simulink model "NearSpace_CMG_AttitudeValidation_S07_sequential"  (R2024a)
settings: Solver=ode4  StartTime=0.0  StopTime=90  FixedStep=.001  RelTol=1e-3
InitFcn:
  | init_paths;
model workspace (MAT data in the model file):
  disturbance_schedule = [0 0.2 0.4 0.6 0.8 1 1.2 1.4 1.6 1.8 2 2.2 ... (1804 elements, 451x4)]
  native_controller_template.N = 22
  native_controller_template.nx = 11
  native_controller_template.nu = 7
  native_controller_template.A = [0.0129318474981 0.00454610585776 -0.104555464036 -0.0430961443461 0 0 0 0 0 0 0 0.0045632886618 ... (2662 elements, 11x11x22)]
  native_controller_template.B = [3.81382167025e-08 8.27941674815e-06 3.61487373465e-07 -8.73828707523e-07 0.000166666673675 6.80437440218e-11 5.83929378418e-08 0 0 0 0 -1.23300542093e-07 ... (1694 elements, 11x7x22)]
  native_controller_template.Q = [2.93800357151 1.03345970786 -23.6701188526 -9.7565805888 0 0 0 0 0 0 0 1.03345970786 ... (2783 elements, 11x11x23)]
  native_controller_template.q = [-8.33060992209e-17 -3.43379209732e-17 7.86467691392e-16 -3.63722284202e-18 0 0 0 0 0 0 0 -4.73641230657e-05 ... (253 elements, 11x23)]
  native_controller_template.R = [4.31034482759e-09 0 0 0 0 0 0 0 4.31034482759e-09 0 0 0 ... (1078 elements, 7x7x22)]
  native_controller_template.r = [0  0  0  0  0  0  0  0  0  0  0  0  0  0  0  0  0  0  0  0  0  0; 0  0  0  0  0  0  0  0  0  0  0  0  0  0  0  0  0  0  0  0  0  0; 0  0  0  0  0  0  0  0  0  0  0  0  0  0  0  0  0  0  0  0  0  0; 0  0  0  0  0  0  0  0  0  0  0  0  0  0  0  0  0  0  0  0  0  0; 0  0  0  0  0  0  0  0  0  0  0  0  0  0  0  0  0  0  0  0  0  0; 0  0  0  0  0  0  0  0  0  0  0  0  0  0  0  0  0  0  0  0  0  0; 0  0  0  0  0  0  0  0  0  0  0  0  0  0  0  0  0  0  0  0  0  0]
  native_controller_template.lu = [-7.49356523213  -7.33777259666  -7.18600471837  -7.03824308743  -6.89428580738  -6.75412475019  -6.61755652855  -6.29144837489  -5.98588397606  -5.69947563015  -5.43093373011  -4.94268279296  -4.51241818721  -4.13264174567  -3.79695534964  -3.2357799895  -2.79208095619  -2.43956912968  -2.15906876065  -1.93640270229  -1.76086736642  -1.62445125088; -40.0303246112  -39.1980515883  -38.3872802015  -37.5979115099  -36.8288669329  -36.0801029921  -35.3505331481  -33.6084121671  -31.9760422139  -30.4460095447  -29.0114244992  -26.4031327314  -24.1046185829  -22.0758239062  -20.2825675451  -17.2847500763  -14.9145096796  -13.0314021867  -11.5329854696  -10.3435215557  -9.40582937798  -8.69691379499; -5.88780125381  -5.76539275452  -5.64614656443  -5.53004814012  -5.41693884866  -5.30681230372  -5.199508701  -4.94328086598  -4.70319455262  -4.47815942369  -4.26716221651  -3.88353648019  -3.54547143281  -3.24707565731  -2.98332206043  -2.54239856318  -2.19377789415  -1.91680431618  -1.69641116908  -1.52145926608  -1.38353864504  -1.27635455426; -0.6  -0.6  -0.6  -0.6  -0.6  -0.6  -1  -1  -1  -1  -1  -1  -1  -1  -1  -1  -1  -1  -1  -1  -1  -1; -0.6  -0.6  -0.6  -0.6  -0.6  -0.6  -1  -1  -1  -1  -1  -1  -1  -1  -1  -1  -1  -1  -1  -1  -1  -1; -0.6  -0.6  -0.6  -0.6  -0.6  -0.6  -1  -1  -1  -1  -1  -1  -1  -1  -1  -1  -1  -1  -1  -1  -1  -1; -0.6  -0.6  -0.6  -0.6  -0.6  -0.6  -1  -1  -1  -1  -1  -1  -1  -1  -1  -1  -1  -1  -1  -1  -1  -1]
  native_controller_template.uu = [7.49356523213  7.33777259666  7.18600471837  7.03824308743  6.89428580738  6.75412475019  6.61755652855  6.29144837489  5.98588397606  5.69947563015  5.43093373011  4.94268279296  4.51241818721  4.13264174567  3.79695534964  3.2357799895  2.79208095619  2.43956912968  2.15906876065  1.93640270229  1.76086736642  1.62445125088; 34.0818590032  33.3733257413  32.683096134  32.011086058  31.356377316  30.7189329988  30.0978281232  28.6147036285  27.2250080988  25.9224307534  24.7011068974  22.480543243  20.5236931588  18.7964570949  17.2697381107  14.7174696001  12.6994777992  11.0962045903  9.8204418335  8.80771396137  8.0093423778  7.36908758731; 5.88780125381  5.76539275452  5.64614656443  5.53004814012  5.41693884866  5.30681230372  5.199508701  4.94328086598  4.70319455262  4.47815942369  4.26716221651  3.88353648019  3.54547143281  3.24707565731  2.98332206043  2.54239856318  2.19377789415  1.91680431618  1.69641116908  1.52145926608  1.38353864504  1.27635455426; 0.6  0.6  0.6  0.6  0.6  0.6  1  1  1  1  1  1  1  1  1  1  1  1  1  1  1  1; 0.6  0.6  0.6  0.6  0.6  0.6  1  1  1  1  1  1  1  1  1  1  1  1  1  1  1  1; 0.6  0.6  0.6  0.6  0.6  0.6  1  1  1  1  1  1  1  1  1  1  1  1  1  1  1  1; 0.6  0.6  0.6  0.6  0.6  0.6  1  1  1  1  1  1  1  1  1  1  1  1  1  1  1  1]
  native_controller_template.tr_J = [0  0  0  0  0  0  0  1  0  0  0; 0  0  0  0  0  0  0  0  1  0  0; 0  0  0  0  0  0  0  0  0  1  0; 0  0  0  0  0  0  0  0  0  0  1; 0  0  0  0  1  0  0  0  0  0  0; 0  0  0  0  0  1  0  0  0  0  0; 0  0  0  0  0  0  1  0  0  0  0]
  native_controller_template.tr_bound = [0.5 0.5 0.5 0.5 1 1 1]
  native_controller_template.dX_python = [3.23606232306e-13 -5.05417641364e-12 -2.92224535378e-12 -6.74312649502e-13 3.78845337087e-12 2.01635192376e-12 2.06409029592e-13 -1.11347932545e-13 5.50085421801e-15 1.26375661699e-13 9.48095246948e-15 2.09238232721e-07 ... (253 elements, 11x23)]
  native_controller_template.dU_python = [-0.246446738654 -0.306453966669 0.13796942633 0.00603294344725 -0.0229922476874 0.00440926582071 0.0232611456455 -0.246916325329 -0.301698755455 0.137744299807 0.00603262858184 -0.0229919425529 ... (154 elements, 7x22)]
  native_controller_template.status_python = 0
  native_controller_template.objective_python = -100.014666684
  native_controller_template.residuals_python = [2.98405715596e-07 5.55111512313e-17 5.130568831e-12 1.67492029611e-07]
  native_controller_template.time_python = 0.00536040001316
  native_controller_template.b = [0  0  0  0  0  0  0  0  0  0  0  0  0  0  0  0  0  0  0  0  0  0; 0  0  0  0  0  0  0  0  0  0  0  0  0  0  0  0  0  0  0  0  0  0; 0  0  0  0  0  0  0  0  0  0  0  0  0  0  0  0  0  0  0  0  0  0; 0  0  0  0  0  0  0  0  0  0  0  0  0  0  0  0  0  0  0  0  0  0; 0  0  0  0  0  0  0  0  0  0  0  0  0  0  0  0  0  0  0  0  0  0; 0  0  0  0  0  0  0  0  0  0  0  0  0  0  0  0  0  0  0  0  0  0; 0  0  0  0  0  0  0  0  0  0  0  0  0  0  0  0  0  0  0  0  0  0; 0  0  0  0  0  0  0  0  0  0  0  0  0  0  0  0  0  0  0  0  0  0; 0  0  0  0  0  0  0  0  0  0  0  0  0  0  0  0  0  0  0  0  0  0; 0  0  0  0  0  0  0  0  0  0  0  0  0  0  0  0  0  0  0  0  0  0; 0  0  0  0  0  0  0  0  0  0  0  0  0  0  0  0  0  0  0  0  0  0]
  native_controller_template.dts = [0.2 0.2 0.2 0.2 0.2 0.2 0.5 0.5 0.5 0.5 1 1 1 1 2 2 2 2 2 2 2 2]
  native_controller_template.X_nom = [0.99349030067 -0.00459465233533 0.105234839865 0.0433767232977 0 -0.00432732065041 -6.93889390391e-15 0 0 0 0 0.993535677662 ... (253 elements, 11x23)]
  native_controller_template.U_nom = [0  0  0  0  0  0  0  0  0  0  0  0  0  0  0  0  0  0  0  0  0  0; 0  0  0  0  0  0  0  0  0  0  0  0  0  0  0  0  0  0  0  0  0  0; 0  0  0  0  0  0  0  0  0  0  0  0  0  0  0  0  0  0  0  0  0  0; 0  0  0  0  0  0  0  0  0  0  0  0  0  0  0  0  0  0  0  0  0  0; 0  0  0  0  0  0  0  0  0  0  0  0  0  0  0  0  0  0  0  0  0  0; 0  0  0  0  0  0  0  0  0  0  0  0  0  0  0  0  0  0  0  0  0  0; 0  0  0  0  0  0  0  0  0  0  0  0  0  0  0  0  0  0  0  0  0  0]
  native_controller_template.q_ref = [0.99349030067  0.99353588687  0.993581565542  0.993627332245  0.993673182524  0.993719111908  0.993765115914  0.993880422829  0.993996097282  0.994112068092  0.99422826362  0.994461040259  0.994693846693  0.994926098112  0.995157206991  0.995613643427  0.996058465484  0.996487049594  0.996894897629  0.997277696515  0.997631377894  0.997927911665  0.997867448535; -0.00459465233533  -0.00457582315754  -0.0045568768741  -0.00453781386592  -0.00451863451821  -0.00449933922046  -0.00447992836644  -0.00443089829597  -0.00438115483786  -0.00433070450158  -0.00427955396824  -0.00417517990016  -0.00406808955824  -0.00395834267937  -0.00384600183703  -0.00361380283738  -0.00337205036695  -0.00312134796667  -0.00286234432899  -0.00259573213135  -0.00232224625292  -0.0020651359066  -0.00212009923104; 0.105234839865  0.104803580791  0.104369639557  0.103933024888  0.103493745604  0.103051810628  0.102607228979  0.10148425574  0.100344943238  0.0991894405636  0.0980179007403  0.0956273415558  0.0931745694718  0.0906609526886  0.0880879243743  0.0827696929255  0.0772326510222  0.0714906220237  0.06555846343  0.059452040163  0.0531881837227  0.0472993886305  0.0485582557271; 0.0433767232977  0.0433787136342  0.0433807080081  0.0433827062255  0.0433847080919  0.0433867134121  0.0433887219904  0.043393756399  0.0433988068547  0.0434038702496  0.0434089434559  0.0434191067035  0.0434292712519  0.0434394115678  0.0434495019994  0.0434694304446  0.043488851795  0.0435075641814  0.0435253712112  0.0435420845715  0.043557526634  0.043570473578  0.0435678337008]
  native_controller_template.omega_ref = [0  -8.67361737988e-16  -8.67361737988e-16  -8.67361737988e-16  8.67361737988e-16  0  0  0  -1.73472347598e-15  -1.73472347598e-15  8.67361737988e-16  -8.67361737988e-16  -8.67361737988e-16  0  0  0  -4.33680868994e-16  4.33680868994e-16  8.67361737988e-16  0  -4.33680868994e-16  4.33680868994e-16  4.33680868994e-16; -0.00432732065041  -0.00435416179159  -0.00438091274321  -0.00440757254696  -0.00443414024177  -0.00446061486409  -0.00448699544751  -0.00455252912383  -0.00461745379622  -0.00468175417555  -0.00474541489068  -0.00487075547607  -0.00499335121638  -0.00511307694423  -0.00522980693007  -0.00545377571478  -0.00566425202773  -0.0058602418583  -0.00604077445642  -0.00620491478813  -0.00635177642281  -0.003982213943  0.00759649136201; -6.93889390391e-15  0  0  0  -6.93889390391e-15  0  0  -6.93889390391e-15  6.93889390391e-15  6.93889390391e-15  0  0  6.93889390391e-15  0  -6.93889390391e-15  -6.93889390391e-15  0  0  -6.93889390391e-15  0  0  0  6.93889390391e-15]
  native_controller_template.tau_d = [0.199484155849  0.199489053409  0.199494626016  0.199500828488  0.199507629621  0.199514985574  0.199522867559  0.199544628593  0.199568924155  0.19959526788  0.19962320929  0.199682264218  0.199743188232  0.199803599356  0.199861590815  0.199964815888  0.200045323596  0.200100167269  0.200129801571  0.200136972413  0.200125756163  0.200100827269  0.200066931025; 0.5  0.499833255306  0.499674052661  0.499522707906  0.499379500971  0.499244655382  0.499118370443  0.498840962593  0.498619137626  0.498452772511  0.498340491986  0.498267419783  0.498370159105  0.498609407079  0.498941211307  0.499708773556  0.500371977343  0.500745449074  0.500779834318  0.500539969817  0.500158481461  0.49978358111  0.499535212067; 0.299521786173  0.299499936275  0.299480381724  0.299463069288  0.299447955631  0.299434979588  0.2994240929  0.299405603066  0.299398796878  0.299402622464  0.299415980939  0.299466794994  0.299542254488  0.299633719845  0.299733257458  0.299929839333  0.300090045125  0.300190786191  0.300226297867  0.300204273637  0.300140997478  0.300056604423  0.299971095849]
  native_controller_template.tau_min = [-7.49356523213  -7.33777259666  -7.18600471837  -7.03824308743  -6.89428580738  -6.75412475019  -6.61755652855  -6.29144837489  -5.98588397606  -5.69947563015  -5.43093373011  -4.94268279296  -4.51241818721  -4.13264174567  -3.79695534964  -3.2357799895  -2.79208095619  -2.43956912968  -2.15906876065  -1.93640270229  -1.76086736642  -1.62445125088  -1.52107277557; -40.0303246112  -39.1980515883  -38.3872802015  -37.5979115099  -36.8288669329  -36.0801029921  -35.3505331481  -33.6084121671  -31.9760422139  -30.4460095447  -29.0114244992  -26.4031327314  -24.1046185829  -22.0758239062  -20.2825675451  -17.2847500763  -14.9145096796  -13.0314021867  -11.5329854696  -10.3435215557  -9.40582937798  -8.69691379499  -8.4168151472; -5.88780125381  -5.76539275452  -5.64614656443  -5.53004814012  -5.41693884866  -5.30681230372  -5.199508701  -4.94328086598  -4.70319455262  -4.47815942369  -4.26716221651  -3.88353648019  -3.54547143281  -3.24707565731  -2.98332206043  -2.54239856318  -2.19377789415  -1.91680431618  -1.69641116908  -1.52145926608  -1.38353864504  -1.27635455426  -1.19512860938]
  native_controller_template.tau_max = [7.49356523213  7.33777259666  7.18600471837  7.03824308743  6.89428580738  6.75412475019  6.61755652855  6.29144837489  5.98588397606  5.69947563015  5.43093373011  4.94268279296  4.51241818721  4.13264174567  3.79695534964  3.2357799895  2.79208095619  2.43956912968  2.15906876065  1.93640270229  1.76086736642  1.62445125088  1.52107277557; 34.0818590032  33.3733257413  32.683096134  32.011086058  31.356377316  30.7189329988  30.0978281232  28.6147036285  27.2250080988  25.9224307534  24.7011068974  22.480543243  20.5236931588  18.7964570949  17.2697381107  14.7174696001  12.6994777992  11.0962045903  9.8204418335  8.80771396137  8.0093423778  7.36908758731  6.62676175404; 5.88780125381  5.76539275452  5.64614656443  5.53004814012  5.41693884866  5.30681230372  5.199508701  4.94328086598  4.70319455262  4.47815942369  4.26716221651  3.88353648019  3.54547143281  3.24707565731  2.98332206043  2.54239856318  2.19377789415  1.91680431618  1.69641116908  1.52145926608  1.38353864504  1.27635455426  1.19512860938]
  native_controller_template.weights.e_scale = 0.0174532925199
  native_controller_template.weights.omega_scale = 0.02
  native_controller_template.weights.d_scale = 20
  native_controller_template.weights.nu_scale = 1.5
  native_controller_template.weights.w_att = 1
  native_controller_template.weights.w_rate = 1
  native_controller_template.weights.q_terminal = 10
  native_controller_template.weights.r_nu = 0.05
  native_controller_template.weights.r_dnu = 0.1
  native_controller_template.weights.r_dtau = 0.0001
  native_controller_template.gdot = 1
  native_controller_template.gddot = 3
  native_controller_template.dt_ctrl = 0.2
  native_controller_template.J = [1200  0  0; 0  8500  0; 0  0  9000]
  native_controller_template.tau_nom = [-0.199484155839  -0.199489053409  -0.199494625995  -0.199500828499  -0.199507629611  -0.199514985574  -0.19952286758  -0.199544628593  -0.199568924155  -0.19959526788  -0.19962320928  -0.199682264218  -0.199743188243  -0.199803599366  -0.19986159082  -0.199964815909  -0.20004532359  -0.200100167264  -0.200129801561  -0.200136972413  -0.200125756169  -0.200100827264  -0.200066931014; -1.64265105641  -1.63867158176  -1.6346589716  -1.63061344696  -1.62653515066  -1.62242419921  -1.61828070145  -1.60777968548  -1.59707508214  -1.58616530152  -1.57504763847  -1.5521731719  -1.52841375407  -1.50372413656  -1.47805680671  -1.42361393458  -1.36480966918  -1.3015319516  -1.23385635195  -1.16202667843  -1.08640977158  32.1226332503  60.0838160682; -0.299521786173  -0.299499936275  -0.299480381099  -0.299463068663  -0.299447955631  -0.299434979588  -0.299424093524  -0.299405602442  -0.299398796878  -0.299402622464  -0.299415981564  -0.29946679437  -0.299542254488  -0.299633719221  -0.299733257458  -0.299929838709  -0.300090045125  -0.300190786815  -0.300226298491  -0.300204273637  -0.300140997478  -0.300056605048  -0.299971097098]
  native_controller_template.gap = [0  0  0  0  0  0  0  0  0  0  0  0  0  0  0  0  0  0  0  0  0  0  0; 0  0  0  0  0  0  0  0  0  0  0  0  0  0  0  0  0  0  0  0  0  24.753545663  53.4570543142; 0  0  0  0  0  0  0  0  0  0  0  0  0  0  0  0  0  0  0  0  0  0  0]
  native_controller_template.h0 = 50
  native_controller_template.s0 = [0  -1  -1.22464679915e-16  1; 1  6.12323399574e-17  -1  -1.83697019872e-16; 0  0  0  0]
  native_controller_template.gxs0 = [-0.577350416216  -3.53525169603e-17  0.577350416216  1.06057550881e-16; 0  -0.577350416216  -7.07050339205e-17  0.577350416216; 0.816496476964  0.816496476964  0.816496476964  0.816496476964]
  native_controller_template.online_command_python = [-0.200489714742 -0.567815829111 -0.297267374811 4.16789170609e-05 -0.0185899464278 6.88875630175e-06 0.0185965034114]
  native_reference_bank.time = [0 0.2 0.4 0.6 0.8 1 1.2 1.4 1.6 1.8 2 2.2 ... (451 elements, 1x451)]
  native_reference_bank.x0 = [0.99349030067 -0.00459465233533 0.105234839865 0.0433767232977 0 -0.00432732065041 -6.93889390391e-15 0 0 0 0]
  native_reference_bank.q_ref = [0.99349030067 -0.00459465233533 0.105234839865 0.0433767232977 0.99353588687 -0.00457582315754 0.104803580791 0.0433787136342 0.993581565542 -0.0045568768741 0.104369639557 0.0433807080081 ... (41492 elements, 4x23x451)]
  native_reference_bank.omega_ref = [0 -0.00432732065041 -6.93889390391e-15 -8.67361737988e-16 -0.00435416179159 0 -8.67361737988e-16 -0.00438091274321 0 -8.67361737988e-16 -0.00440757254696 0 ... (31119 elements, 3x23x451)]
  native_reference_bank.tau_d = [0.199484155849 0.5 0.299521786173 0.199489053409 0.499833255306 0.299499936275 0.199494626016 0.499674052661 0.299480381724 0.199500828488 0.499522707906 0.299463069288 ... (31119 elements, 3x23x451)]
  native_reference_bank.tau_min = [-7.49356523213 -40.0303246112 -5.88780125381 -7.33777259666 -39.1980515883 -5.76539275452 -7.18600471837 -38.3872802015 -5.64614656443 -7.03824308743 -37.5979115099 -5.53004814012 ... (31119 elements, 3x23x451)]
  native_reference_bank.tau_max = [7.49356523213 34.0818590032 5.88780125381 7.33777259666 33.3733257413 5.76539275452 7.18600471837 32.683096134 5.64614656443 7.03824308743 32.011086058 5.53004814012 ... (31119 elements, 3x23x451)]
  native_reference_bank.tau_nom = [-0.199484155839 -1.64265105641 -0.299521786173 -0.199489053409 -1.63867158176 -0.299499936275 -0.199494625995 -1.6346589716 -0.299480381099 -0.199500828499 -1.63061344696 -0.299463068663 ... (31119 elements, 3x23x451)]
  native_reference_bank.gap = [0 0 0 0 0 0 0 0 0 0 0 0 ... (31119 elements, 3x23x451)]
  reference_attitude_deg = [0 0.2 0.4 0.6 0.8 1 1.2 1.4 1.6 1.8 2 2.2 ... (1804 elements, 451x4)]
  reference_body_rate = [0 0.2 0.4 0.6 0.8 1 1.2 1.4 1.6 1.8 2 2.2 ... (1804 elements, 451x4)]
  reference_torque_nom = [0 0.2 0.4 0.6 0.8 1 1.2 1.4 1.6 1.8 2 2.2 ... (1804 elements, 451x4)]
  reference_window = [-1e-06 0.199999 0.399999 0.599999 0.799999 0.999999 1.199999 1.399999 1.599999 1.799999 1.999999 2.199999 ... (194832 elements, 451x432)]
libraries: aerolibprivatev1p5 x1
(part 1 of 2)
settings Model: Creator=zz  LastModifiedBy=zz

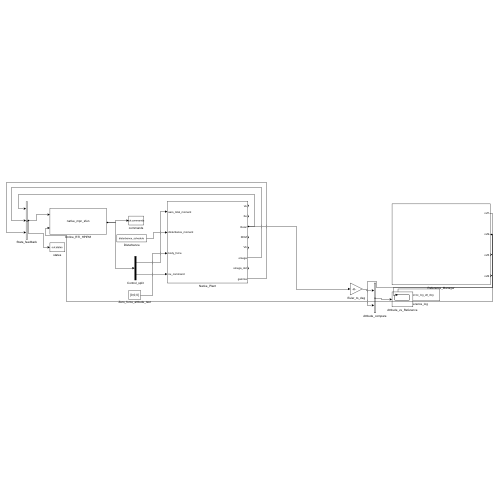
[thumbnail: Simulink's stored preview of the top-level diagram]
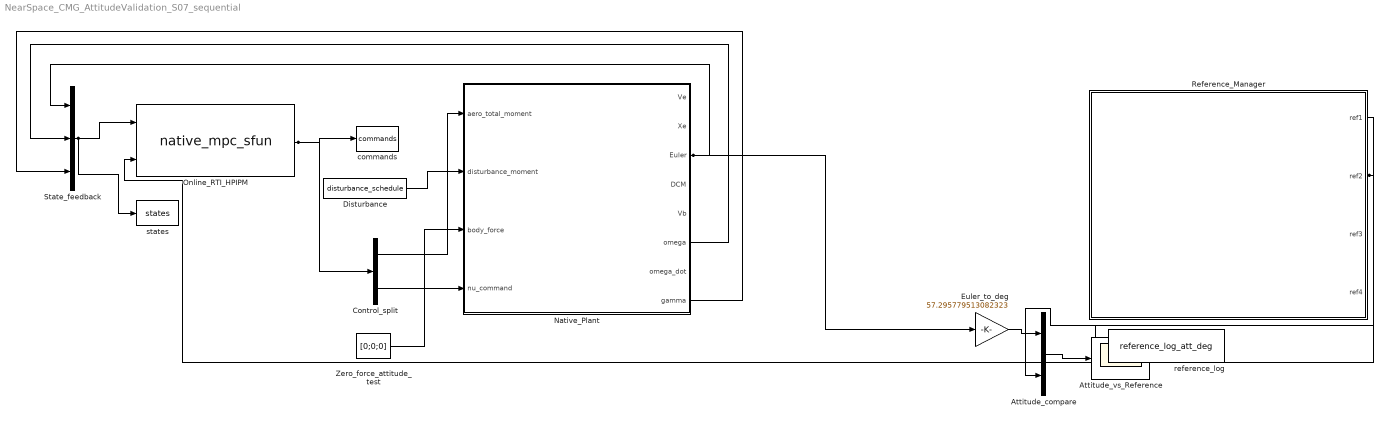
== system NearSpace_CMG_AttitudeValidation_S07_sequential ==
  Attitude_compare : Mux  Inputs=2
  Attitude_vs_Reference : Scope
  Control_split : Demux  Outputs=[3 4]
  Disturbance : FromWorkspace  VariableName=disturbance_schedule  Interpolate=off  OutputAfterFinalValue=Holding final value
  Euler_to_deg : Gain  Gain=57.295779513082323
  Native_Plant : Subsystem
  Online_RTI_HPIPM : M-S-Function  FunctionName=native_mpc_sfun
  Reference_Manager : Subsystem
  State_feedback : Mux  Inputs=3
  Zero_force_attitude_test : Constant  Value=[0;0;0]
  commands : ToWorkspace  VariableName=commands  SaveFormat=Timeseries
  reference_log : ToWorkspace  VariableName=reference_log_att_deg  SaveFormat=Timeseries
  states : ToWorkspace  VariableName=states  SaveFormat=Timeseries
  wires:
  State_feedback/1 -> states/1, Online_RTI_HPIPM/1
  Disturbance/1 -> Native_Plant/2(disturbance_moment)
  Zero_force_attitude_test/1 -> Native_Plant/3(body_force)
  Control_split/2 -> Native_Plant/4(nu_command)
  Control_split/1 -> Native_Plant/1(aero_total_moment)
  Native_Plant/3(Euler) -> State_feedback/1, Euler_to_deg/1
  Native_Plant/6(omega) -> State_feedback/2
  Native_Plant/8(gamma) -> State_feedback/3
  Online_RTI_HPIPM/1 -> Control_split/1, commands/1
  Reference_Manager/1(ref1) -> Online_RTI_HPIPM/2
  Reference_Manager/2(ref2) -> reference_log/1, Attitude_compare/2
  Euler_to_deg/1 -> Attitude_compare/1
  Attitude_compare/1 -> Attitude_vs_Reference/1
